simulink model "FOCwithLOAD"  (R2024b)
settings: Solver=FixedStepDiscrete  StartTime=0.0  StopTime=inf  RelTol=1e-3
PreLoadFcn:
  | % 自动加载同目录下的 linear_data.m，确保换机/首次打开可直接更新与编译
  | if ~evalin('base', 'exist(''Ts'',''var'') && exist(''pmsm'',''var'') && exist(''SMRC_I_Vsat_thresh'',''var'')')
  |     mdlDir_ = '';
  |     if bdIsLoaded('FOCwithLOAD'), mdlDir_ = fileparts(get_param('FOCwithLOAD', 'FileName')); end
  |     if isempty(mdlDir_), mdlDir_ = fileparts(which('FOCwithLOAD')); end
  |     if isempty(mdlDir_), mdlDir_ = pwd; end
  |     dataFile_ = fullfile(mdlDir_, 'linear_data.m');
  |     if isfile(dataFile_)
  |         assignin('base', 'linearDataFileTmp_', dataFile_);
  |         evalin('base', 'run(linearDataFileTmp_); clear linearDataFileTmp_');
  |     end
  |     clear mdlDir_ dataFile_
  | end
InitFcn:
  | % 自动加载同目录下的 linear_data.m，确保换机/首次打开可直接更新与编译
  | if ~evalin('base', 'exist(''Ts'',''var'') && exist(''pmsm'',''var'') && exist(''SMRC_I_Vsat_thresh'',''var'')')
  |     mdlDir_ = '';
  |     if bdIsLoaded('FOCwithLOAD'), mdlDir_ = fileparts(get_param('FOCwithLOAD', 'FileName')); end
  |     if isempty(mdlDir_), mdlDir_ = fileparts(which('FOCwithLOAD')); end
  |     if isempty(mdlDir_), mdlDir_ = pwd; end
  |     dataFile_ = fullfile(mdlDir_, 'linear_data.m');
  |     if isfile(dataFile_)
  |         assignin('base', 'linearDataFileTmp_', dataFile_);
  |         evalin('base', 'run(linearDataFileTmp_); clear linearDataFileTmp_');
  |     end
  |     clear mdlDir_ dataFile_
  | end
values from neighbouring files (symbols this model uses):
  a_hat = Kt_eff / (pmsm.J * omega_pu_base)    [linear_data.m]
  ADRC_B0 = 6055    [linear_data.m]
  ADRC_Wc = 3.2e-3    (= 0.0032)    [linear_data.m]
  ADRC_Wo = 30    [linear_data.m]
  alpha_ppc = exp(-lambda_ppc*Ts_speed)    [linear_data.m]
  b_hat = pmsm.B/pmsm.J    [linear_data.m]
  beta1 = single(2.0 * w_o)    [linear_data.m]
  beta2_sat_scale = 0.2    [linear_data.m]
  dataType = 'single'    [linear_data.m]
  gamma_reset = 0.9    [linear_data.m]
  inv_a_hat = 1/double(a_hat)    [linear_data.m]
  k_xi = 55    [linear_data.m]
  Kff = 0.98931745    [linear_data.m]
  lambda_ppc = 45    [linear_data.m]
  P_inf_const = 0.004    [linear_data.m]
  PI_params = mcb_SetControllerParameters(pmsm,inverter,PU_System,T_pwm,Ts,Ts_speed)    [linear_data.m]
  pmsm2 = pmsm    [linear_data.m]
  s_limit_sat = 0.9    [linear_data.m]
  speedRPM2mmps = pmlsm.mmps_per_rpm    [linear_data.m]
  target = mcb_SetProcessorDetails('F28379D',PWM_frequency)    [linear_data.m]
  Ts = T_pwm    (= 5e-05)    [linear_data.m]
  Ts_motor = T_pwm/2    (= 2.5e-05)    [linear_data.m]
  Ts_speed = 1*Ts    (= 5e-05)    [linear_data.m]
  w_o = single(200.0)    [linear_data.m]
  z2_limit = single(100.0)    [linear_data.m]
undefined symbols (not defined in the file or in its folder): DiscIntNeverNeededParam, Down, GPTRIP1SEL, GPTRIP2SEL, innerPI, inverter, inverter2, outerPI, pmlsm, pmsm, Tctr, TZ1, TZ2, Up
libraries: c2802xlib x13, simulink x10, c2837xDlib x6, c280xlib x6, slpidlib x5, svdschedulerlib x4, mcbcontrolslib x4, mcbpositiondecoderlib x2, mcbpmsmnonlinearlib x2, autolibpmsmexterior x2, mcbplantlib x2, svdutilitieslib x1
(part 3 of 5)

== system FOCwithLOAD/Motor1 Speed control/SCI (Code Generation)/Data_Conditioning_Tx ==
  In1 : Inport
  Data_Type_Fixed_Point : Subsystem  VariantControl=~isequal(dataType,'single')
  Data_Type_Float : Subsystem  VariantControl=isequal(dataType, 'single')
  Data_Log : Outport

== system FOCwithLOAD/Motor1 Speed control/SCI (Code Generation)/Data_Logging ==
  note: Fast Serial Data Monitoring (32-bit)
  Data_Log : Inport
  Counter Limited : simulink/Sources/Counter Limited  uplimit=600-1  tsamp=-1
  Data : Subsystem  TreatAsAtomicUnit=on
  End : Subsystem  TreatAsAtomicUnit=on
  If : If  IfExpression=u1 == 0  ElseIfExpressions=u1 == 599
  Merge : Merge  Inputs=3
  Merge1 : Merge  Inputs=3
  Mux : Mux  Inputs=2
  Start : Subsystem  TreatAsAtomicUnit=on
  Width : Width  OutDataTypeMode=All ports same datatype  DataType=uint16
  SCI_Tx : Outport
  wires:
  If/3 -> Data/Action
  Data/1(Data_out) -> Merge/3
  Width/1 -> Data/2(Data_width), Start/2(Data_width), End/2(Data_width)
  Merge/1 -> Mux/1  "SCI_Tx_Data"
  Counter Limited/1 -> If/1
  Start/2(Iteration) -> Merge1/1
  Start/1(Data_out) -> Merge/1
  If/2 -> End/Action
  Merge1/1 -> Mux/2  "SCI_Tx_Iteration"
  If/1 -> Start/Action
  End/1(Data_out) -> Merge/2
  End/2(Iteration) -> Merge1/2
  Data/2(Iteration) -> Merge1/3
  Mux/1 -> SCI_Tx/1
  Data_Log/1 -> Width/1, Start/1(Data), End/1(Data), Data/1(Data)

== system FOCwithLOAD/Motor1 Speed control/SCI (Code Generation)/While Iterator Subsystem ==
  Data : Inport
  Iteration : Inport  Port=2
  Add : Sum  Inputs=+-  OutDataTypeStr=Inherit: Same as first input
  Index Vector : MultiPortSwitch  Inputs=1  SaturateOnIntegerOverflow=off  InputSameDT=off
  SCI Transmit : c280xlib/SCI Transmit  sciModule=A  dataHead=''  dataTail=''  frameSize=1  blockingMode=on  outputStatus=off
  While Iterator : WhileIterator  MaxIters=-1  WhileBlockType=do-while  ShowIterationPort=on  OutputDataType=int16
  wires:
  While Iterator/1 -> Add/2, Index Vector/1
  Data/1 -> Index Vector/2
  Index Vector/1 -> SCI Transmit/1
  Add/1 -> While Iterator/1
  Iteration/1 -> Add/1

== system FOCwithLOAD/Motor1 and Motor2 coupled/Simulation/Load_Friction ==
  spd_rpm : Inport
  Fc_to_Tq : Gain  Gain=pmlsm.F_fric_rated*pmlsm.tau_elec/(2*pi)
  inv_veps : Gain  Gain=1/0.002
  rpm2mps : Gain  Gain=pmlsm.rpm2mps
  tanh_fric : Trigonometry  Operator=tanh
  T_fric : Outport
  wires:
  spd_rpm/1 -> rpm2mps/1
  rpm2mps/1 -> inv_veps/1
  inv_veps/1 -> tanh_fric/1
  tanh_fric/1 -> Fc_to_Tq/1
  Fc_to_Tq/1 -> T_fric/1

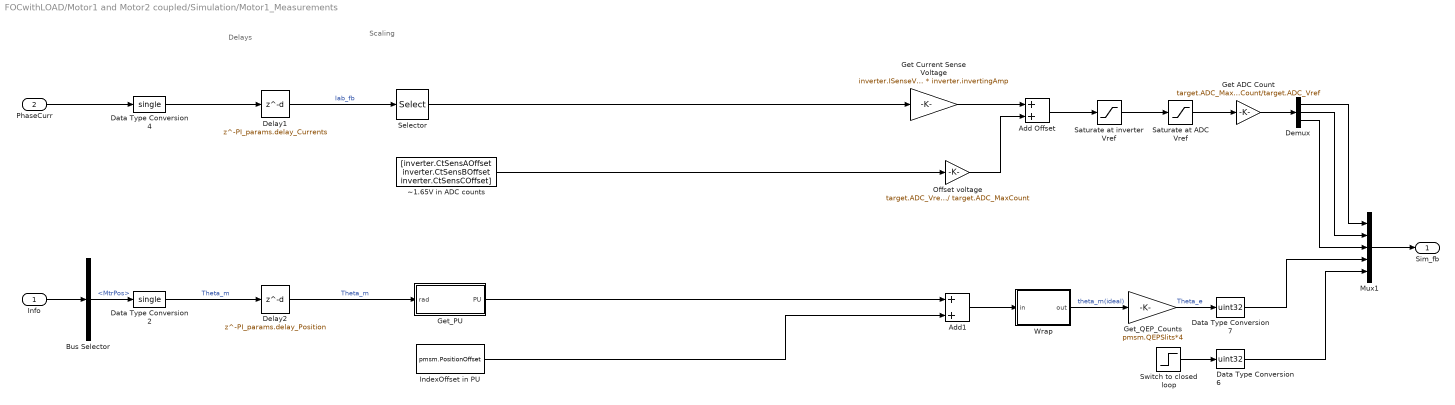
== system FOCwithLOAD/Motor1 and Motor2 coupled/Simulation/Motor1_Measurements ==
  note: Delays
  note: Scaling
  Info : Inport
  PhaseCurr : Inport  Port=2
  Add Offset : Sum  RndMeth=Simplest
  Add1 : Sum  RndMeth=Simplest
  Bus Selector : BusSelector  OutputSignals=MtrPos
  Data Type Conversion2 : DataTypeConversion  OutDataTypeStr=single  RndMeth=Simplest  SaturateOnIntegerOverflow=off
  Data Type Conversion4 : DataTypeConversion  OutDataTypeStr=single  RndMeth=Simplest  SaturateOnIntegerOverflow=off
  Data Type Conversion6 : DataTypeConversion  OutDataTypeStr=uint32  RndMeth=Simplest  SaturateOnIntegerOverflow=off
  Data Type Conversion7 : DataTypeConversion  OutDataTypeStr=uint32  RndMeth=Simplest  SaturateOnIntegerOverflow=off
  Delay1 : Delay  DelayLength=PI_params.delay_Currents
  Delay2 : Delay  DelayLength=PI_params.delay_Position
  Demux : Demux  Outputs=3
  Get ADC Count : Gain  Gain=target.ADC_MaxCount/target.ADC_Vref  OutMin=0  OutMax=target.ADC_MaxCount  OutDataTypeStr=uint32  RndMeth=Simplest
  Get Current Sense Voltage : Gain  Gain=inverter.ISenseVoltPerAmp * inverter.invertingAmp  RndMeth=Simplest  OutDataTypeStr=Inherit: Same as input
  "Get_PU " : Subsystem
  Get_QEP_Counts : Gain  Gain=pmsm.QEPSlits*4  OutDataTypeStr=uint32  RndMeth=Simplest
  IndexOffset in PU : Constant  Value=pmsm.PositionOffset  OutDataTypeStr=single  SampleTime=-1
  Mux1 : Mux  Inputs=5
  Offset voltage : Gain  Gain=target.ADC_Vref / target.ADC_MaxCount  RndMeth=Simplest
  Saturate at ADC Vref : Saturate  UpperLimit=target.ADC_Vref  LowerLimit=0
  Saturate at inverter Vref : Saturate  UpperLimit=inverter.ISenseVref  LowerLimit=0
  Selector : Selector  InputPortWidth=3  IndexOptions=Index vector (dialog)  Indices=[1 2 3]  OutputSizes=1
  "Switch to closed loop " : Step  Time=0.1  SampleTime=Ts_motor
  Wrap : Subsystem
  ~1.65V in ADC counts : Constant  Value="[inverter.CtSensAOffset inverter.CtSensBOffset  inverter.CtSensCOffset]"  OutDataTypeStr=uint16  SampleTime=-1
  Sim_fb : Outport  VectorParamsAs1DForOutWhenUnconnected=off
  wires:
  "Switch to closed loop "/1 -> Data Type Conversion6/1
  Data Type Conversion6/1 -> Mux1/5
  Data Type Conversion7/1 -> Mux1/4
  IndexOffset in PU/1 -> Add1/2
  Get_QEP_Counts/1 -> Data Type Conversion7/1  "Theta_e"
  "Get_PU "/1(PU) -> Add1/1
  Wrap/1(out) -> Get_QEP_Counts/1  "theta_m(ideal)"
  Delay2/1 -> "Get_PU "/1(rad)  "Theta_m"
  Add1/1 -> Wrap/1(in)
  Data Type Conversion2/1 -> Delay2/1  "Theta_m"
  Demux/2 -> Mux1/2
  Mux1/1 -> Sim_fb/1
  Demux/1 -> Mux1/1
  Bus Selector/1 -> Data Type Conversion2/1  "<MtrPos>"
  Info/1 -> Bus Selector/1
  PhaseCurr/1 -> Data Type Conversion4/1
  Data Type Conversion4/1 -> Delay1/1
  Delay1/1 -> Selector/1  "Iab_fb"
  Saturate at ADC Vref/1 -> Get ADC Count/1
  Offset voltage/1 -> Add Offset/2
  Get ADC Count/1 -> Demux/1
  Saturate at inverter Vref/1 -> Saturate at ADC Vref/1
  Add Offset/1 -> Saturate at inverter Vref/1
  Get Current Sense Voltage/1 -> Add Offset/1
  ~1.65V in ADC counts/1 -> Offset voltage/1
  Demux/3 -> Mux1/3
  Selector/1 -> Get Current Sense Voltage/1

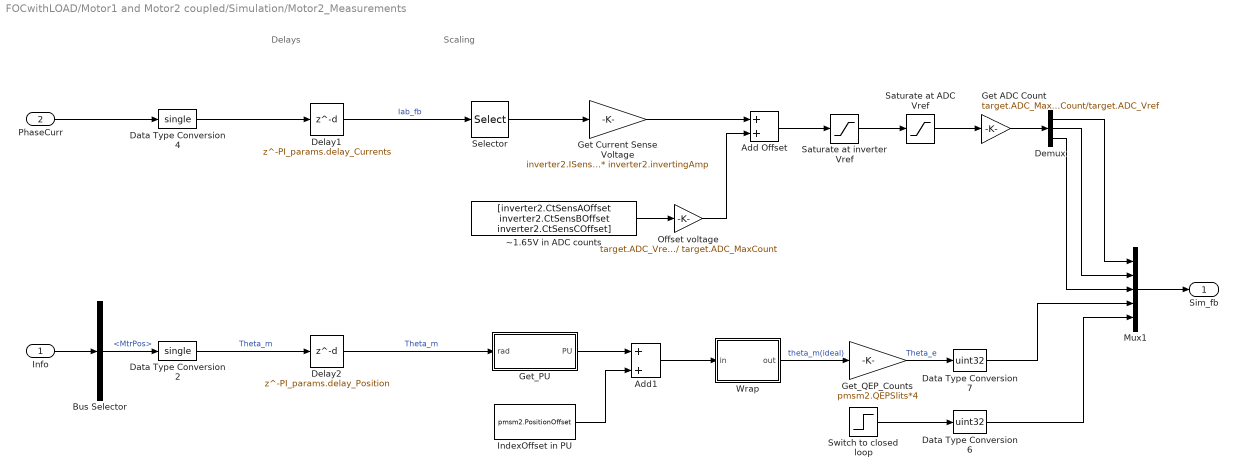
== system FOCwithLOAD/Motor1 and Motor2 coupled/Simulation/Motor2_Measurements ==
  note: Scaling
  note: Delays
  Info : Inport
  PhaseCurr : Inport  Port=2
  Add Offset : Sum  RndMeth=Simplest
  Add1 : Sum  RndMeth=Simplest
  Bus Selector : BusSelector  OutputSignals=MtrPos
  Data Type Conversion2 : DataTypeConversion  OutDataTypeStr=single  RndMeth=Simplest  SaturateOnIntegerOverflow=off
  Data Type Conversion4 : DataTypeConversion  OutDataTypeStr=single  RndMeth=Simplest  SaturateOnIntegerOverflow=off
  Data Type Conversion6 : DataTypeConversion  OutDataTypeStr=uint32  RndMeth=Simplest  SaturateOnIntegerOverflow=off
  Data Type Conversion7 : DataTypeConversion  OutDataTypeStr=uint32  RndMeth=Simplest  SaturateOnIntegerOverflow=off
  Delay1 : Delay  DelayLength=PI_params.delay_Currents
  Delay2 : Delay  DelayLength=PI_params.delay_Position
  Demux : Demux  Outputs=3
  Get ADC Count : Gain  Gain=target.ADC_MaxCount/target.ADC_Vref  OutMin=0  OutMax=target.ADC_MaxCount  OutDataTypeStr=uint32  RndMeth=Simplest
  Get Current Sense Voltage : Gain  Gain=inverter2.ISenseVoltPerAmp * inverter2.invertingAmp  RndMeth=Simplest  OutDataTypeStr=Inherit: Same as input
  "Get_PU " : Subsystem
  Get_QEP_Counts : Gain  Gain=pmsm2.QEPSlits*4  OutDataTypeStr=uint32  RndMeth=Simplest
  IndexOffset in PU : Constant  Value=pmsm2.PositionOffset  OutDataTypeStr=single  SampleTime=-1
  Mux1 : Mux  Inputs=5
  Offset voltage : Gain  Gain=target.ADC_Vref / target.ADC_MaxCount  RndMeth=Simplest
  Saturate at ADC Vref : Saturate  UpperLimit=target.ADC_Vref  LowerLimit=0
  Saturate at inverter Vref : Saturate  UpperLimit=inverter2.ISenseVref  LowerLimit=0
  Selector : Selector  InputPortWidth=3  IndexOptions=Index vector (dialog)  Indices=[1 2 3]  OutputSizes=1
  "Switch to closed loop " : Step  Time=0.1  SampleTime=Ts_motor
  Wrap : Subsystem
  ~1.65V in ADC counts : Constant  Value=[inverter2.CtSensAOffset inverter2.CtSensBOffset inverter2.CtSensCOffset]  OutDataTypeStr=uint16  SampleTime=-1
  Sim_fb : Outport  VectorParamsAs1DForOutWhenUnconnected=off
  wires:
  Delay1/1 -> Selector/1  "Iab_fb"
  Data Type Conversion4/1 -> Delay1/1
  PhaseCurr/1 -> Data Type Conversion4/1
  Info/1 -> Bus Selector/1
  Bus Selector/1 -> Data Type Conversion2/1  "<MtrPos>"
  Demux/1 -> Mux1/1
  Mux1/1 -> Sim_fb/1
  Demux/2 -> Mux1/2
  Data Type Conversion2/1 -> Delay2/1  "Theta_m"
  Add1/1 -> Wrap/1(in)
  Delay2/1 -> "Get_PU "/1(rad)  "Theta_m"
  Wrap/1(out) -> Get_QEP_Counts/1  "theta_m(ideal)"
  "Get_PU "/1(PU) -> Add1/1
  Get_QEP_Counts/1 -> Data Type Conversion7/1  "Theta_e"
  IndexOffset in PU/1 -> Add1/2
  Data Type Conversion7/1 -> Mux1/4
  Data Type Conversion6/1 -> Mux1/5
  "Switch to closed loop "/1 -> Data Type Conversion6/1
  Saturate at ADC Vref/1 -> Get ADC Count/1
  Offset voltage/1 -> Add Offset/2
  Selector/1 -> Get Current Sense Voltage/1
  Get ADC Count/1 -> Demux/1
  Saturate at inverter Vref/1 -> Saturate at ADC Vref/1
  Add Offset/1 -> Saturate at inverter Vref/1
  Get Current Sense Voltage/1 -> Add Offset/1
  ~1.65V in ADC counts/1 -> Offset voltage/1
  Demux/3 -> Mux1/3

== system FOCwithLOAD/Motor1 and Motor2 coupled/Simulation/Mtr1 Inverter ==
  Duty_abc : Inport
  Average-Value Inverter : mcbplantlib/Average-Value Inverter
  Constant2 : Constant  Value=inverter.V_dc  OutDataTypeStr=single
  Data Type Conversion1 : DataTypeConversion  OutDataTypeStr=single  RndMeth=Simplest  SaturateOnIntegerOverflow=off
  Rate Transition3 : RateTransition  Integrity=off  OutPortSampleTime=Ts_inverter
  Vabc : Outport  VectorParamsAs1DForOutWhenUnconnected=off
  wires:
  Constant2/1 -> Average-Value Inverter/2
  Data Type Conversion1/1 -> Rate Transition3/1
  Average-Value Inverter/1 -> Vabc/1
  Duty_abc/1 -> Data Type Conversion1/1
  Rate Transition3/1 -> Average-Value Inverter/1

== system FOCwithLOAD/Motor1 and Motor2 coupled/Simulation/Mtr2 Inverter ==
  Duty_abc : Inport
  Average-Value Inverter : mcbplantlib/Average-Value Inverter
  Constant2 : Constant  Value=inverter2.V_dc  OutDataTypeStr=single
  Data Type Conversion1 : DataTypeConversion  OutDataTypeStr=single  RndMeth=Simplest  SaturateOnIntegerOverflow=off
  Rate Transition3 : RateTransition  Integrity=off  OutPortSampleTime=Ts_inverter
  Vabc : Outport  VectorParamsAs1DForOutWhenUnconnected=off
  wires:
  Data Type Conversion1/1 -> Rate Transition3/1
  Average-Value Inverter/1 -> Vabc/1
  Duty_abc/1 -> Data Type Conversion1/1
  Rate Transition3/1 -> Average-Value Inverter/1
  Constant2/1 -> Average-Value Inverter/2

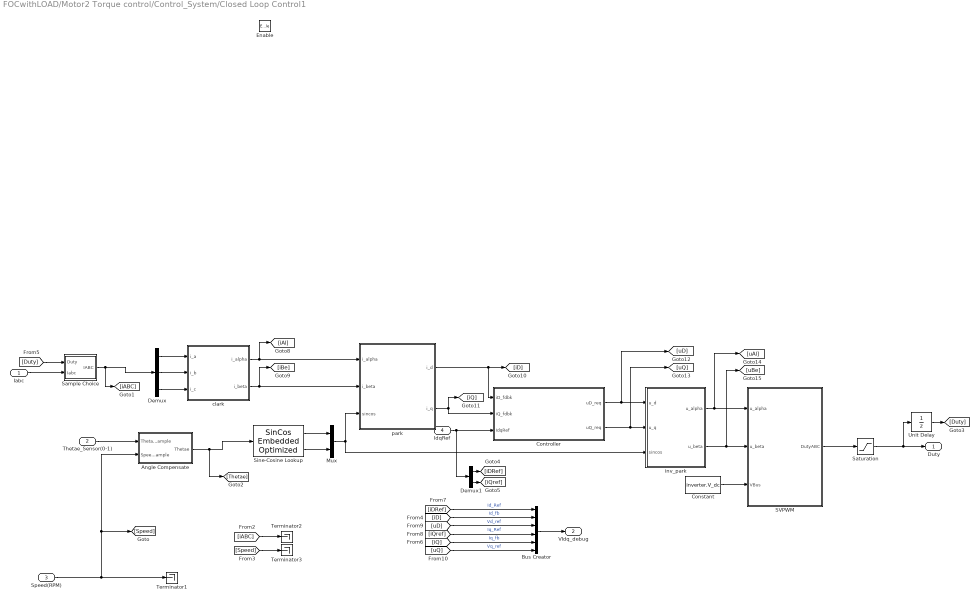
== system FOCwithLOAD/Motor2 Torque control/Control_System/Closed Loop Control1 ==
  Iabc : Inport
  Thetae_Sensor(0-1) : Inport  Port=2
  Speed(RPM) : Inport  Port=3
  IdqRef : Inport  Port=4
  Enable : EnablePort
  Angle Compensate : Subsystem
  Bus Creator : BusCreator  Inputs=6
  Constant : Constant  Value=inverter.V_dc  OutDataTypeStr=single
  Controller : Subsystem
  Demux : Demux  Outputs=3
  Demux1 : Demux  Outputs=2
  Mux : Mux  Inputs=2
  SVPWM : Subsystem
      mask Display:
      | port_label('input',1,'u_{\alpha}','texmode','on');
      | port_label('input',2,'u_{\beta}','texmode','on');
      | port_label('input',3,'V_{Bus}','texmode','on');
      | 
      | port_label('output',1,'Duty_{ABC}','texmode','on');
      | 
      | fprintf('SVPWM');
  Sample Choice : Subsystem
  Saturation : Saturate  UpperLimit=1  LowerLimit=0
  Sine-Cosine Lookup : mcbcontrolslib/SinCos Embedded Optimized  LabelModeActiveChoice=MCB_Sin  OptforProc=off  ApproximationMethod=None  UserApproxMethod=Lookup  ApproxStatus=None  InterpMethod=Linear point-slope  NumberOfDataPoints=16  NumberOfIterations=11  RemoveProtectionAgainstOutOfRangeInput=off  TableDataTypeStr=Inherit: Inherit via input  AngleInput=Per-unit  ThetaDataType=single  N_points=1024  DatatypeInput=Inherit from input  Datatype=Inherit: Same as input
  Terminator1 : Terminator
  Terminator2 : Terminator
  Terminator3 : Terminator
  Unit Delay : UnitDelay  SampleTime=-1  HasFrameUpgradeWarning=on
  clark : Subsystem  TreatAsAtomicUnit=on
      mask Display:
      | port_label('input',1,'a','texmode','on');
      | port_label('input',2,'b','texmode','on');
      | port_label('input',3,'c','texmode','on');
      | 
      | port_label('output',1,'\alpha','texmode','on');
      | port_label('output',2,'\beta','texmode','on');
      | 
      | fprintf('Clark');
  inv_park : Subsystem
      mask Display:
      | port_label('input', 1, 'd', 'texmode', 'on');
      | port_label('input', 2, 'q', 'texmode', 'on');
      | port_label('input', 3, 'sin\theta_e cos\theta_e', 'texmode', 'on');
      | port_label('output', 1, '\alpha', 'texmode', 'on');
      | port_label('output', 2, '\beta', 'texmode', 'on');
      | fprintf('Inverse Park')
  park : Subsystem  TreatAsAtomicUnit=on
      mask Display:
      | port_label('input',1,'\alpha','texmode','on');
      | port_label('input',2,'\beta','texmode','on');
      | port_label('input',3,'sin\theta_e cos\theta_e','texmode','on');
      | 
      | port_label('output',1,'d','texmode','on');
      | port_label('output',2,'q','texmode','on');
      | 
      | fprintf('Park');
  Duty : Outport
  VIdq_debug : Outport  Port=2  VectorParamsAs1DForOutWhenUnconnected=off
  wires:
  inv_park/2(u_beta) -> [uBe], SVPWM/2(u_beta)
  Saturation/1 -> Unit Delay/1, Duty/1
  Demux/2 -> clark/2(i_b)
  Demux/3 -> clark/3(i_c)
  Mux/1 -> inv_park/3(sincos), park/3(sincos)
  Controller/2(uQ_req) -> inv_park/2(u_q), [uQ]
  SVPWM/1(DutyABC) -> Saturation/1
  park/1(i_d) -> [iD], Controller/1(iD_fdbk)
  Controller/1(uD_req) -> inv_park/1(u_d), [uD]
  clark/1(i_alpha) -> [iAl], park/1(i_alpha)
  clark/2(i_beta) -> [iBe], park/2(i_beta)
  inv_park/1(u_alpha) -> [uAl], SVPWM/1(u_alpha)
  park/2(i_q) -> Controller/2(iQ_fdbk), [iQ]
  Demux/1 -> clark/1(i_a)
  Sine-Cosine Lookup/1 -> Mux/1
  Sine-Cosine Lookup/2 -> Mux/2
  [Duty] -> Sample Choice/1(Duty)
  Unit Delay/1 -> [Duty]
  Constant/1 -> SVPWM/3(VBus)
  Speed(RPM)/1 -> Terminator1/1, Angle Compensate/2(SpeedSample), [Speed]
  Thetae_Sensor(0-1)/1 -> Angle Compensate/1(ThetaeSample)
  Angle Compensate/1(Thetae) -> [Thetae], Sine-Cosine Lookup/1
  Iabc/1 -> Sample Choice/2(Iabc)
  Sample Choice/1(IABC) -> Demux/1, [iABC]
  [iABC] -> Terminator2/1
  [Speed] -> Terminator3/1
  IdqRef/1 -> Demux1/1, Controller/3(IdqRef)
  [iDRef] -> Bus Creator/1  "Id_Ref"
  [iD] -> Bus Creator/2  "Id_fb"
  Bus Creator/1 -> VIdq_debug/1
  [uQ] -> Bus Creator/6  "Vq_ref"
  [uD] -> Bus Creator/3  "Vd_ref"
  [iQ] -> Bus Creator/5  "Iq_fb"
  [iQref] -> Bus Creator/4  "Iq_Ref"
  Demux1/1 -> [iDRef]
  Demux1/2 -> [iQref]

== system FOCwithLOAD/Motor2 Torque control/HW_Inputs/Sensor Driver Blocks (codegen) ==
  Sim : Inport
  ADC_A_IN4 : c2802xlib/ADC  Priority=1  blkParamProc=C2000_Type4  ADCModule=A  samplingMode=Single sample mode  ADCResolution=12-bit (Single-ended input)  useSOC1=SOC1  useSOC2=SOC0_SOC1  SOCAcquisitionWindow=30  SOCTriggerSource=ePWM4_ADCSOCA  SOCInterruptTrigger=No ADCINT  Ts=-1  dType=uint16  postInterrupt=off  interruptSel=ADCINT1  ADCINTContinuous=on  endma=off  chdma=1  conv1=ADCINA0  conv2=ADCINA0 and ADCINB0  conv1_Type4=ADCIN4  conv2_Type4=ADCIN0 and ADCIN1
  ADC_A_IN4_u32 : DataTypeConversion  OutDataTypeStr=uint32  SaturateOnIntegerOverflow=off  RndMeth=Floor
  ADC_B_IN4 : c2802xlib/ADC  Priority=2  blkParamProc=C2000_Type4  ADCModule=B  samplingMode=Single sample mode  ADCResolution=12-bit (Single-ended input)  useSOC1=SOC1  useSOC2=SOC0_SOC1  SOCAcquisitionWindow=30  SOCTriggerSource=ePWM4_ADCSOCA  SOCInterruptTrigger=No ADCINT  Ts=-1  dType=uint16  postInterrupt=off  interruptSel=ADCINT1  ADCINTContinuous=on  endma=off  chdma=1  conv1=ADCINA0  conv2=ADCINA0 and ADCINB0  conv1_Type4=ADCIN4  conv2_Type4=ADCIN0 and ADCIN1
  ADC_B_IN4_u32 : DataTypeConversion  OutDataTypeStr=uint32  SaturateOnIntegerOverflow=off  RndMeth=Floor
  ADC_C_IN4 : c2802xlib/ADC  Priority=3  blkParamProc=C2000_Type4  ADCModule=C  samplingMode=Single sample mode  ADCResolution=12-bit (Single-ended input)  useSOC1=SOC1  useSOC2=SOC0_SOC1  SOCAcquisitionWindow=30  SOCTriggerSource=ePWM4_ADCSOCA  SOCInterruptTrigger=No ADCINT  Ts=-1  dType=uint16  postInterrupt=on  interruptSel=ADCINT1  ADCINTContinuous=on  endma=off  chdma=1  conv1=ADCINA0  conv2=ADCINA0 and ADCINB0  conv1_Type4=ADCIN4  conv2_Type4=ADCIN0 and ADCIN1
  ADC_C_IN4_u32 : DataTypeConversion  OutDataTypeStr=uint32  SaturateOnIntegerOverflow=off  RndMeth=Floor
  Mux1 : Mux  Inputs=5
  Terminator : Terminator
  eQEP2 for PMSM2 : c280xlib/eQEP  Priority=0  useModule=eQEP2  pcInputmode=Quadrature-count  externalClockrate=2x resolution: Count the rising/falling edge  swapPolarityselection=Counterclockwise  qdfOutputport=off  qapPolarityselection=off  qbpPolarityselection=off  qipPolarityselection=off  qspPolarityselection=off  igatePolarityselection=off  sampleTime=-1  pcOutputport=on  pcMaximumvalue=2^32-1  indexInitializationcheck=off  indexInitializationevent=Rising edge  strobeInitializationcheck=off  strobeInitializationevent=Rising edge  softwareInitializationcheck=off  softwareInitializationsource=Set to init value at start up  softwareInitializationmode=on  pcInitialvalue=0  pcResetmode=Reset on the maximum position  ieloutputport=on  indexEventlatch=Rising edge  seloutputport=off  strobeEventlatch=Rising edge  pcefOutputport=off  enableEqepcapture=off  qctmrOutputport=off  qcprdOutputport=off  captureTimerprescaler=128  upEventprescaler=128  overflowErrorflag=off  directionErrorflag=off  captureTimerposition=On position counter read  unitTimerperiod=100000000  captureTimerlatch=off  capturePeriodlatch=off  positionCounterlatch=off  soenPolarityselection=off  spselPolarityselection=Index pin is used for sync output  compareValuesource=Specify via dialog  shadowMode=Load on QPOSCNT=0  compareValue=4294967295  syncOutputwidth=1  polaritySyncoutput=Active high  watchdogEnable=off  watchdogTimer=65535  outport1Datatype=uint32  outport2Datatype=auto  outport3Datatype=auto  outport4Datatype=auto  outport5Datatype=auto  outport6Datatype=auto  outport7Datatype=auto  outport8Datatype=auto  outport9Datatype=auto  outport10Datatype=auto  outport11Datatype=auto  outport12Datatype=auto  eqepinterrupt_pce=off  eqepinterrupt_qpe=off  eqepinterrupt_qdc=off  eqepinterrupt_wto=off  eqepinterrupt_pcu=off  eqepinterrupt_pco=off  eqepinterrupt_pcr=off  eqepinterrupt_pcm=off  eqepinterrupt_sel=off  eqepinterrupt_iel=off  eqepinterrupt_uto=off  pheOutputport=off  watchdogOutputport=off  outport13Datatype=auto  outport14Datatype=auto
      settings: LibrarySourceBlock=c28002xlib/eQEP
  read_qep32 : CFunction  OutputCode=|  CodegenOutputCode=|
      OutputCode=|
      | /* 32-bit read: legacy c280xqep truncates QPOSCNT to uint16 */
      | y1 = (uint32_T)EQep2Regs.QPOSCNT;
      | y2 = (uint32_T)EQep2Regs.QPOSILAT;
      CodegenOutputCode=|
      | /* 32-bit read: legacy c280xqep truncates QPOSCNT to uint16 */
      | y1 = (uint32_T)EQep2Regs.QPOSCNT;
      | y2 = (uint32_T)EQep2Regs.QPOSILAT;
  term_qep2_1 : Terminator
  term_qep2_2 : Terminator
  Out : Outport
  wires:
  Mux1/1 -> Out/1
  Sim/1 -> Terminator/1
  ADC_A_IN4/1 -> ADC_A_IN4_u32/1
  ADC_A_IN4_u32/1 -> Mux1/1
  ADC_B_IN4/1 -> ADC_B_IN4_u32/1
  ADC_B_IN4_u32/1 -> Mux1/2
  ADC_C_IN4/1 -> ADC_C_IN4_u32/1
  ADC_C_IN4_u32/1 -> Mux1/3
  eQEP2 for PMSM2/1 -> term_qep2_1/1
  eQEP2 for PMSM2/2 -> term_qep2_2/1
  read_qep32/1 -> Mux1/4
  read_qep32/2 -> Mux1/5

== system FOCwithLOAD/Motor2 Torque control/HW_Inputs/Sensor Driver Blocks (sim) ==
  Sim : Inport
  Out : Outport
  wires:
  Sim/1 -> Out/1

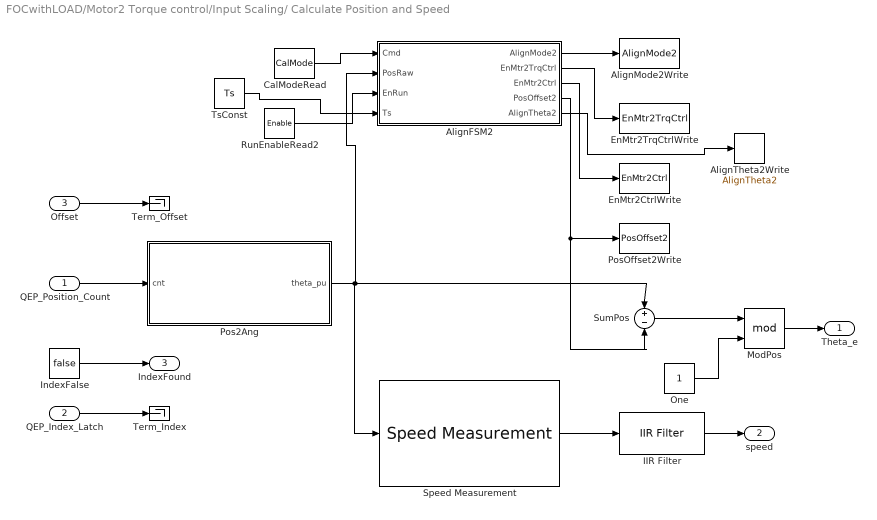
== system FOCwithLOAD/Motor2 Torque control/Input Scaling/ Calculate Position and Speed ==
  QEP_Position_Count : Inport
  QEP_Index_Latch : Inport  Port=2
  Offset : Inport  Port=3
  AlignFSM2 : MATLAB Function  TreatAsAtomicUnit=on
  AlignMode2Write : DataStoreWrite  DataStoreName=AlignMode2  IndexOptions=Index vector (dialog)  Indices=1  OutputSizes=1
  AlignTheta2Write : DataStoreWrite  DataStoreName=AlignTheta2  IndexOptions=Index vector (dialog)  Indices=1  OutputSizes=1
  CalModeRead : DataStoreRead  DataStoreName=CalMode  IndexOptions=Index vector (dialog)  Indices=1  OutputSizes=1
  EnMtr2CtrlWrite : DataStoreWrite  DataStoreName=EnMtr2Ctrl  IndexOptions=Index vector (dialog)  Indices=1  OutputSizes=1
  EnMtr2TrqCtrlWrite : DataStoreWrite  DataStoreName=EnMtr2TrqCtrl  IndexOptions=Index vector (dialog)  Indices=1  OutputSizes=1
  IIR Filter : mcbcontrolslib/IIR Filter  VariantControl=Low Pass Filter  VariantSelect=Low-pass  FilterConstantInputType=Specify via dialog  Filter_constant=0.1  advancedSettings=on  Ts=50e-6  cutOff_freq=353.6777
  IndexFalse : Constant  Value=false  OutDataTypeStr=boolean
  ModPos : Math  Operator=mod
  One : Constant  OutDataTypeStr=single
  Pos2Ang : MATLAB Function  TreatAsAtomicUnit=on
  PosOffset2Write : DataStoreWrite  DataStoreName=PosOffset2  IndexOptions=Index vector (dialog)  Indices=1  OutputSizes=1
  RunEnableRead2 : DataStoreRead  DataStoreName=Enable  IndexOptions=Index vector (dialog)  Indices=1  OutputSizes=1
  Speed Measurement : mcbpositiondecoderlib/Speed Measurement  PositionUnit=Per unit  PositionScalingDatatype=uint32  SpeedCalculationMode=Time interval for speed calculation  SampleTimeAsync=Ts  MaximumApplicationSpeed=6000  SpeedResolution=5e-6  DelayLength=200  MaximumMeasurableSpeed=2999  MeasurableSpeedResolution=1.397e-06  SpeedUnit=RPM  PerUnitSpeed=3000  SpeedDataType=dataType
  SumPos : Sum  Inputs=+-
  Term_Index : Terminator
  Term_Offset : Terminator
  TsConst : Constant  Value=Ts  OutDataTypeStr=single
  Theta_e : Outport  VectorParamsAs1DForOutWhenUnconnected=off
  speed : Outport  Port=2  VectorParamsAs1DForOutWhenUnconnected=off
  IndexFound : Outport  Port=3
  wires:
  CalModeRead/1 -> AlignFSM2/1(Cmd)
  ModPos/1 -> Theta_e/1
  Offset/1 -> Term_Offset/1
  QEP_Position_Count/1 -> Pos2Ang/1(cnt)
  QEP_Index_Latch/1 -> Term_Index/1
  IndexFalse/1 -> IndexFound/1
  AlignFSM2/1(AlignMode2) -> AlignMode2Write/1
  Pos2Ang/1(theta_pu) -> SumPos/1, AlignFSM2/2(PosRaw), Speed Measurement/1
  AlignFSM2/2(EnMtr2TrqCtrl) -> EnMtr2TrqCtrlWrite/1
  AlignFSM2/3(EnMtr2Ctrl) -> EnMtr2CtrlWrite/1
  AlignFSM2/4(PosOffset2) -> SumPos/2, PosOffset2Write/1
  Speed Measurement/1 -> IIR Filter/1
  SumPos/1 -> ModPos/1
  One/1 -> ModPos/2
  IIR Filter/1 -> speed/1
  RunEnableRead2/1 -> AlignFSM2/3(EnRun)
  AlignFSM2/5(AlignTheta2) -> AlignTheta2Write/1
  TsConst/1 -> AlignFSM2/4(Ts)

== system FOCwithLOAD/Motor2 Torque control/Input Scaling/Calculate Phase Currents ==
  Ia_ADC : Inport
  Ib_ADC : Inport  Port=2
  Ic_ADC : Inport  Port=3
  Add : Sum  Inputs=-+
  Data Store Read1 : DataStoreRead  DataStoreName=IaOffset_motor2  IndexOptions=Index vector (dialog)  Indices=1  OutputSizes=1
  Data Store Read2 : DataStoreRead  DataStoreName=IbOffset_motor2  IndexOptions=Index vector (dialog)  Indices=1  OutputSizes=1
  Data Store Read4 : DataStoreRead  DataStoreName=IcOffset_motor2  IndexOptions=Index vector (dialog)  Indices=1  OutputSizes=1
  Data Type Conversion : DataTypeConversion  OutDataTypeStr=int32  ConvertRealWorld=Stored Integer (SI)  RndMeth=Simplest  SaturateOnIntegerOverflow=off
  Data_Type : Subsystem  Variant=on
  Inverting / Non-inverting Current measurement amplifieer : Gain  Gain=inverter2.invertingAmp  RndMeth=Simplest  OutDataTypeStr=Inherit: Same as input
  Mux : Mux  Inputs=3
  Mux1 : Mux  Inputs=3
  Iabc_meas_Real : Outport  VectorParamsAs1DForOutWhenUnconnected=off
  wires:
  Data Type Conversion/1 -> Add/2
  Data_Type/1(Iabc_meas_Real) -> Inverting / Non-inverting Current measurement amplifieer/1
  Ia_ADC/1 -> Mux/1
  Ib_ADC/1 -> Mux/2
  Mux/1 -> Data Type Conversion/1
  Data Store Read1/1 -> Mux1/1
  Data Store Read2/1 -> Mux1/2
  Mux1/1 -> Add/1
  Add/1 -> Data_Type/1(In1)
  Ic_ADC/1 -> Mux/3
  Data Store Read4/1 -> Mux1/3
  Inverting / Non-inverting Current measurement amplifieer/1 -> Iabc_meas_Real/1

== system FOCwithLOAD/Motor2 Torque control/Inverter/Code Generation ==
  note: for inverter connected with LaunchXL-28379D
  note: System Outputs
  Inverter Signals : Inport
  Constant : Constant  Value=inverter2.EnableLogic
  Demux : Demux
  Demux1 : Demux  Outputs=3
  Ground : Ground
  Ground1 : Ground
  Ground2 : Ground
  Inverter2 Enable : c2837xDlib/Digital Output  GPIO_Number=GPIO8~GPIO15  GPIO_Bit0=off  GPIO_BIT0_Toggle=off  GPIO_Bit1=off  GPIO_BIT1_Toggle=off  GPIO_Bit2=off  GPIO_BIT2_Toggle=off  GPIO_Bit3=off  GPIO_BIT3_Toggle=off  GPIO_Bit4=off  GPIO_BIT4_Toggle=off  GPIO_Bit5=off  GPIO_BIT5_Toggle=off  GPIO_Bit6=on  GPIO_BIT6_Toggle=off  GPIO_Bit7=off  GPIO_BIT7_Toggle=off
  Mux : Mux  Inputs=3
  Mux1 : Mux  Inputs=3
  Mux2 : Mux  Inputs=3
  NOT : Logic  Operator=NOT  IconShape=distinctive  AllPortsSameDT=off  OutDataTypeStr=boolean
  Scale_to_PWM_Counter_PRD : Gain  Gain=target.PWM_Counter_Period  OutDataTypeStr=uint16  RndMeth=Simplest
  Switch : Switch  Criteria=u2 > Threshold  SaturateOnIntegerOverflow=off  InputSameDT=off
  Switch1 : Switch  Threshold=0.5  SaturateOnIntegerOverflow=off  InputSameDT=off
  ePWM4 : c2802xlib/ePWM  PwmType=C2000_Type4  useModule=ePWM4  ePWMxLINKTBPRD=Not Linked  periodUnits=Clock cycles  timerSource=Specify via dialog  timerPeriod_clk=target.PWM_Counter_Period  timerPeriod_sec=0.0001  tbshadow=Counter equals to zero  countingMode=Up-Down  phaseActiveEnable=Set counter to phase value specified via dialog  phaseDirection=Count down after sync  phaseActive=target.PWM_Counter_Period  synchronizationEnable=off  dcaevt1Sync=off  dcbevt1Sync=off  synchronizationOption=Pass through (EPWMxSYNCI or SWFSYNC)  dcbevt1SyncOut=off  dcaevt1SyncOut=off  cmpdSyncOut=off  cmpcSyncOut=off  cmpbSyncOut=off  zeroSyncOut=off  swfSyncOut=on  perSynchronizationOption=Counter equals to period (CTR=PRD)  clockPrescale=1  HSclockPrescale=1  enswap=off  ePWMxAStatus=on  ePWMxAactionLogic1=Do nothing  ePWMxAactionLogic2=Do nothing  ePWMxAactionLogic3=Clear  ePWMxAactionLogic4=Set  ePWMxAactionLogic5=Do nothing  ePWMxAactionLogic6=Do nothing  ePWMxACSFenable=off  ePWMxACSFvalue=Forcing disable  ePWMxASFreload=Zero  ePWMxBStatus=off  ePWMxBactionLogic1=Set  ePWMxBactionLogic2=Clear  ePWMxBactionLogic3=Do nothing  ePWMxBactionLogic4=Do nothing  ePWMxBactionLogic5=Clear  ePWMxBactionLogic6=Set  ePWMxBCSFenable=off  ePWMxBCSFvalue=Forcing disable  ePWMxBSFreload=Zero  ePWNxBOutWay=off  ePWMxLINKCMPA=Not Linked  CMPAUnits=Clock cycles  CMPASource=Input port  CMPAValue_per=50  CMPAValue_clk=floor(target.PWM_Counter_Period/2)  enCMPAshadow=Counter equals to zero (CTR=Zero)  ePWMxLINKCMPB=Not Linked  CMPBUnits=Clock cycles  CMPBSource=Specify via dialog  CMPBValue_per=50  CMPBValue_clk=floor(target.PWM_Counter_Period/2)  enCMPBshadow=Counter equals to zero (CTR=Zero)  ePWMxLINKCMPC=Not Linked  CMPCUnits=Clock cycles  CMPCSource=Specify via dialog  CMPCValue_per=50  CMPCValue_clk=32000  enCMPCshadow=Counter equals to zero (CTR=Zero)  ePWMxLINKCMPD=Not Linked  CMPDUnits=Clock cycles  CMPDSource=Specify via dialog  CMPDValue_per=50  CMPDValue_clk=32000  enCMPDshadow=Counter equals to zero (CTR=Zero)  enableDBePWMxA=on  enableDBePWMxB=on  enhalfcycle=off  DBpolarity=Active high complementary (AHC)  DBedgeDelay=Positive  DBSource_ePWMxA=ePWMxA  DBSource_ePWMxB=ePWMxA  DBPeriodUnits=Clock cycles  DBperiodSource=Specify via dialog  REDperiod=10  FEDperiod=10  REDperiod_sec=0  FEDperiod_sec=0  LoadModeDBRED=Immediate without using shadow  LoadModeDBFED=Immediate without using shadow  adcstartModuleA=on  adcrequestEventA=First event  adcstartEventA=Digital Compare Module A Event 1 start of conversion (DCAEVT1.soc)  adcstartEventA_type2=Counter equals to period (CTR=PRD)  adcstartModuleB=off  adcrequestEventB=First event  adcstartEventB=Counter equals to zero (CTR=Zero)  adcstartEventB_type2=Counter equals to zero (CTR=Zero)  intEn=off  intPrd=First event  intSel=Counter equals to zero (CTR=Zero)  intSel_type2=Counter equals to zero (CTR=Zero)  hrpe=off  enHRPWM=off  HRPWM_LoadMode=Counter equals to period (CTR=PRD)  HRPWM_CTLMode=Duty or Period control mode  HRPWM_EDGMode=Both edge  hrpeb=off  enHRPWMB=off  HRPWM_LoadModeB=Counter equals to zero (CTR=ZERO)  HRPWM_CTLModeB=Duty or Period control mode  HRPWM_EDGModeB=Both edge  enHRDBRED=off  enHRDBFED=off  enSFO=on  enautoconv=on  chopperEnable=off  chopperFrequency=1  chopperFirstwidth=1  chopperDuty=12.5%  tripZonesource=Specify via dialog  tzselOSHT1=off  tzselOSHT2=off  tzselOSHT3=off  tzselOSHT4=off  tzselOSHT5=off  tzselOSHT6=off  tzselOSHDCAEV1=off  tzselOSHDCBEV1=off  tzselCBC1=off  tzselCBC2=off  tzselCBC3=off  tzselCBC4=off  tzselCBC5=off  tzselCBC6=off  tzselCBCDCAEV2=off  tzselCBCDCBEV2=off  enTzOstIntr=off  enTzCbcIntr=off  enTzDCAEVT1Intr=off  enTzDCAEVT2Intr=off  enTzDCBEVT1Intr=off  enTzDCBEVT2Intr=off  tzclrCBCLatch=Counter equals to zero (CTR=Zero)  ePWMxAforced=No action  ePWMxBforced=No action  DCAEVT1forced=No action  DCBEVT1forced=No action  DCAEVT2forced=No action  DCBEVT2forced=No action  dcah=Trip Zone 1 input (TZ1)  dcal=Trip Zone 2 input (TZ2)  dcbh=Trip Zone 1 input (TZ1)  dcbl=Trip Zone 2 input (TZ2)  dcah_type2=GPTRIP1SEL/(TZ1)  dcal_type2=GPTRIP2SEL/(TZ2)  dcbh_type2=GPTRIP1SEL/(TZ1)  dcbl_type2=GPTRIP2SEL/(TZ2)  gendcaevt1=Event disabled  gendcaevt2=Event disabled  gendcbevt1=Event disabled  gendcbevt2=Event disabled  dcaevt1src=DCAEVT1 with sync  dcaevt2src=DCAEVT2 with sync  dcbevt1src=DCBEVT1 with sync  dcbevt2src=DCBEVT2 with sync  pulsesel=Counter equals to zero (CTR=Zero)  blankinv=off  blankoffset=0  blankwidth=0  evsrcsel=Filtered version of DCAEVT1 (DCAEVT1FILT)  encape=off
  ePWM5 : c2802xlib/ePWM  PwmType=C2000_Type4  useModule=ePWM5  ePWMxLINKTBPRD=Not Linked  periodUnits=Clock cycles  timerSource=Specify via dialog  timerPeriod_clk=target.PWM_Counter_Period  timerPeriod_sec=0.0001  tbshadow=Counter equals to zero  countingMode=Up-Down  phaseActiveEnable=Set counter to phase value specified via dialog  phaseDirection=Count down after sync  phaseActive=target.PWM_Counter_Period  synchronizationEnable=off  dcaevt1Sync=off  dcbevt1Sync=off  synchronizationOption=Pass through (EPWMxSYNCI or SWFSYNC)  dcbevt1SyncOut=off  dcaevt1SyncOut=off  cmpdSyncOut=off  cmpcSyncOut=off  cmpbSyncOut=off  zeroSyncOut=off  swfSyncOut=on  perSynchronizationOption=Counter equals to period (CTR=PRD)  clockPrescale=1  HSclockPrescale=1  enswap=off  ePWMxAStatus=on  ePWMxAactionLogic1=Do nothing  ePWMxAactionLogic2=Do nothing  ePWMxAactionLogic3=Clear  ePWMxAactionLogic4=Set  ePWMxAactionLogic5=Do nothing  ePWMxAactionLogic6=Do nothing  ePWMxACSFenable=off  ePWMxACSFvalue=Forcing disable  ePWMxASFreload=Zero  ePWMxBStatus=off  ePWMxBactionLogic1=Set  ePWMxBactionLogic2=Clear  ePWMxBactionLogic3=Do nothing  ePWMxBactionLogic4=Do nothing  ePWMxBactionLogic5=Clear  ePWMxBactionLogic6=Set  ePWMxBCSFenable=off  ePWMxBCSFvalue=Forcing disable  ePWMxBSFreload=Zero  ePWNxBOutWay=off  ePWMxLINKCMPA=Not Linked  CMPAUnits=Clock cycles  CMPASource=Input port  CMPAValue_per=50  CMPAValue_clk=floor(target.PWM_Counter_Period/2)  enCMPAshadow=Counter equals to zero (CTR=Zero)  ePWMxLINKCMPB=Not Linked  CMPBUnits=Clock cycles  CMPBSource=Specify via dialog  CMPBValue_per=50  CMPBValue_clk=floor(target.PWM_Counter_Period/2)  enCMPBshadow=Counter equals to zero (CTR=Zero)  ePWMxLINKCMPC=Not Linked  CMPCUnits=Clock cycles  CMPCSource=Specify via dialog  CMPCValue_per=50  CMPCValue_clk=32000  enCMPCshadow=Counter equals to zero (CTR=Zero)  ePWMxLINKCMPD=Not Linked  CMPDUnits=Clock cycles  CMPDSource=Specify via dialog  CMPDValue_per=50  CMPDValue_clk=32000  enCMPDshadow=Counter equals to zero (CTR=Zero)  enableDBePWMxA=on  enableDBePWMxB=on  enhalfcycle=off  DBpolarity=Active high complementary (AHC)  DBedgeDelay=Positive  DBSource_ePWMxA=ePWMxA  DBSource_ePWMxB=ePWMxA  DBPeriodUnits=Clock cycles  DBperiodSource=Specify via dialog  REDperiod=10  FEDperiod=10  REDperiod_sec=0  FEDperiod_sec=0  LoadModeDBRED=Immediate without using shadow  LoadModeDBFED=Immediate without using shadow  adcstartModuleA=off  adcrequestEventA=First event  adcstartEventA=Digital Compare Module A Event 1 start of conversion (DCAEVT1.soc)  adcstartEventA_type2=Counter equals to period (CTR=PRD)  adcstartModuleB=off  adcrequestEventB=First event  adcstartEventB=Counter equals to zero (CTR=Zero)  adcstartEventB_type2=Counter equals to zero (CTR=Zero)  intEn=off  intPrd=First event  intSel=Counter equals to zero (CTR=Zero)  intSel_type2=Counter equals to zero (CTR=Zero)  hrpe=off  enHRPWM=off  HRPWM_LoadMode=Counter equals to period (CTR=PRD)  HRPWM_CTLMode=Duty or Period control mode  HRPWM_EDGMode=Both edge  hrpeb=off  enHRPWMB=off  HRPWM_LoadModeB=Counter equals to zero (CTR=ZERO)  HRPWM_CTLModeB=Duty or Period control mode  HRPWM_EDGModeB=Both edge  enHRDBRED=off  enHRDBFED=off  enSFO=on  enautoconv=on  chopperEnable=off  chopperFrequency=1  chopperFirstwidth=1  chopperDuty=12.5%  tripZonesource=Specify via dialog  tzselOSHT1=off  tzselOSHT2=off  tzselOSHT3=off  tzselOSHT4=off  tzselOSHT5=off  tzselOSHT6=off  tzselOSHDCAEV1=off  tzselOSHDCBEV1=off  tzselCBC1=off  tzselCBC2=off  tzselCBC3=off  tzselCBC4=off  tzselCBC5=off  tzselCBC6=off  tzselCBCDCAEV2=off  tzselCBCDCBEV2=off  enTzOstIntr=off  enTzCbcIntr=off  enTzDCAEVT1Intr=off  enTzDCAEVT2Intr=off  enTzDCBEVT1Intr=off  enTzDCBEVT2Intr=off  tzclrCBCLatch=Counter equals to zero (CTR=Zero)  ePWMxAforced=No action  ePWMxBforced=No action  DCAEVT1forced=No action  DCBEVT1forced=No action  DCAEVT2forced=No action  DCBEVT2forced=No action  dcah=Trip Zone 1 input (TZ1)  dcal=Trip Zone 2 input (TZ2)  dcbh=Trip Zone 1 input (TZ1)  dcbl=Trip Zone 2 input (TZ2)  dcah_type2=GPTRIP1SEL/(TZ1)  dcal_type2=GPTRIP2SEL/(TZ2)  dcbh_type2=GPTRIP1SEL/(TZ1)  dcbl_type2=GPTRIP2SEL/(TZ2)  gendcaevt1=Event disabled  gendcaevt2=Event disabled  gendcbevt1=Event disabled  gendcbevt2=Event disabled  dcaevt1src=DCAEVT1 with sync  dcaevt2src=DCAEVT2 with sync  dcbevt1src=DCBEVT1 with sync  dcbevt2src=DCBEVT2 with sync  pulsesel=Counter equals to zero (CTR=Zero)  blankinv=off  blankoffset=0  blankwidth=0  evsrcsel=Filtered version of DCAEVT1 (DCAEVT1FILT)  encape=off
  ePWM6 : c2802xlib/ePWM  PwmType=C2000_Type4  useModule=ePWM6  ePWMxLINKTBPRD=Not Linked  periodUnits=Clock cycles  timerSource=Specify via dialog  timerPeriod_clk=target.PWM_Counter_Period  timerPeriod_sec=0.0001  tbshadow=Counter equals to zero  countingMode=Up-Down  phaseActiveEnable=Set counter to phase value specified via dialog  phaseDirection=Count down after sync  phaseActive=target.PWM_Counter_Period  synchronizationEnable=off  dcaevt1Sync=off  dcbevt1Sync=off  synchronizationOption=Pass through (EPWMxSYNCI or SWFSYNC)  dcbevt1SyncOut=off  dcaevt1SyncOut=off  cmpdSyncOut=off  cmpcSyncOut=off  cmpbSyncOut=off  zeroSyncOut=off  swfSyncOut=on  perSynchronizationOption=Counter equals to period (CTR=PRD)  clockPrescale=1  HSclockPrescale=1  enswap=off  ePWMxAStatus=on  ePWMxAactionLogic1=Do nothing  ePWMxAactionLogic2=Do nothing  ePWMxAactionLogic3=Clear  ePWMxAactionLogic4=Set  ePWMxAactionLogic5=Do nothing  ePWMxAactionLogic6=Do nothing  ePWMxACSFenable=off  ePWMxACSFvalue=Forcing disable  ePWMxASFreload=Zero  ePWMxBStatus=off  ePWMxBactionLogic1=Set  ePWMxBactionLogic2=Clear  ePWMxBactionLogic3=Do nothing  ePWMxBactionLogic4=Do nothing  ePWMxBactionLogic5=Clear  ePWMxBactionLogic6=Set  ePWMxBCSFenable=off  ePWMxBCSFvalue=Forcing disable  ePWMxBSFreload=Zero  ePWNxBOutWay=off  ePWMxLINKCMPA=Not Linked  CMPAUnits=Clock cycles  CMPASource=Input port  CMPAValue_per=50  CMPAValue_clk=floor(target.PWM_Counter_Period/2)  enCMPAshadow=Counter equals to zero (CTR=Zero)  ePWMxLINKCMPB=Not Linked  CMPBUnits=Clock cycles  CMPBSource=Specify via dialog  CMPBValue_per=50  CMPBValue_clk=floor(target.PWM_Counter_Period/2)  enCMPBshadow=Counter equals to zero (CTR=Zero)  ePWMxLINKCMPC=Not Linked  CMPCUnits=Clock cycles  CMPCSource=Specify via dialog  CMPCValue_per=50  CMPCValue_clk=32000  enCMPCshadow=Counter equals to zero (CTR=Zero)  ePWMxLINKCMPD=Not Linked  CMPDUnits=Clock cycles  CMPDSource=Specify via dialog  CMPDValue_per=50  CMPDValue_clk=32000  enCMPDshadow=Counter equals to zero (CTR=Zero)  enableDBePWMxA=on  enableDBePWMxB=on  enhalfcycle=off  DBpolarity=Active high complementary (AHC)  DBedgeDelay=Positive  DBSource_ePWMxA=ePWMxA  DBSource_ePWMxB=ePWMxA  DBPeriodUnits=Clock cycles  DBperiodSource=Specify via dialog  REDperiod=10  FEDperiod=10  REDperiod_sec=0  FEDperiod_sec=0  LoadModeDBRED=Immediate without using shadow  LoadModeDBFED=Immediate without using shadow  adcstartModuleA=off  adcrequestEventA=First event  adcstartEventA=Digital Compare Module A Event 1 start of conversion (DCAEVT1.soc)  adcstartEventA_type2=Counter equals to period (CTR=PRD)  adcstartModuleB=off  adcrequestEventB=First event  adcstartEventB=Counter equals to zero (CTR=Zero)  adcstartEventB_type2=Counter equals to zero (CTR=Zero)  intEn=off  intPrd=First event  intSel=Counter equals to zero (CTR=Zero)  intSel_type2=Counter equals to zero (CTR=Zero)  hrpe=off  enHRPWM=off  HRPWM_LoadMode=Counter equals to period (CTR=PRD)  HRPWM_CTLMode=Duty or Period control mode  HRPWM_EDGMode=Both edge  hrpeb=off  enHRPWMB=off  HRPWM_LoadModeB=Counter equals to zero (CTR=ZERO)  HRPWM_CTLModeB=Duty or Period control mode  HRPWM_EDGModeB=Both edge  enHRDBRED=off  enHRDBFED=off  enSFO=on  enautoconv=on  chopperEnable=off  chopperFrequency=1  chopperFirstwidth=1  chopperDuty=12.5%  tripZonesource=Specify via dialog  tzselOSHT1=off  tzselOSHT2=off  tzselOSHT3=off  tzselOSHT4=off  tzselOSHT5=off  tzselOSHT6=off  tzselOSHDCAEV1=off  tzselOSHDCBEV1=off  tzselCBC1=off  tzselCBC2=off  tzselCBC3=off  tzselCBC4=off  tzselCBC5=off  tzselCBC6=off  tzselCBCDCAEV2=off  tzselCBCDCBEV2=off  enTzOstIntr=off  enTzCbcIntr=off  enTzDCAEVT1Intr=off  enTzDCAEVT2Intr=off  enTzDCBEVT1Intr=off  enTzDCBEVT2Intr=off  tzclrCBCLatch=Counter equals to zero (CTR=Zero)  ePWMxAforced=No action  ePWMxBforced=No action  DCAEVT1forced=No action  DCBEVT1forced=No action  DCAEVT2forced=No action  DCBEVT2forced=No action  dcah=Trip Zone 1 input (TZ1)  dcal=Trip Zone 2 input (TZ2)  dcbh=Trip Zone 1 input (TZ1)  dcbl=Trip Zone 2 input (TZ2)  dcah_type2=GPTRIP1SEL/(TZ1)  dcal_type2=GPTRIP2SEL/(TZ2)  dcbh_type2=GPTRIP1SEL/(TZ1)  dcbl_type2=GPTRIP2SEL/(TZ2)  gendcaevt1=Event disabled  gendcaevt2=Event disabled  gendcbevt1=Event disabled  gendcbevt2=Event disabled  dcaevt1src=DCAEVT1 with sync  dcaevt2src=DCAEVT2 with sync  dcbevt1src=DCBEVT1 with sync  dcbevt2src=DCBEVT2 with sync  pulsesel=Counter equals to zero (CTR=Zero)  blankinv=off  blankoffset=0  blankwidth=0  evsrcsel=Filtered version of DCAEVT1 (DCAEVT1FILT)  encape=off
  stop : Constant  Value=0  OutDataTypeStr=uint16
  DutyCycles : Outport  VectorParamsAs1DForOutWhenUnconnected=off
  wires:
  Demux1/3 -> ePWM6/1  "PWM_C"
  Scale_to_PWM_Counter_PRD/1 -> Switch1/1
  Mux2/1 -> Switch1/3
  stop/1 -> Mux2/3, Mux2/2, Mux2/1
  Demux/4 -> Switch1/2, NOT/1, Switch/1  "Active high logic for inverter enable"
  Inverter Signals/1 -> Demux/1
  Demux1/2 -> ePWM5/1  "PWM_B"
  Switch1/1 -> Demux1/1
  Demux1/1 -> ePWM4/1  "PWM_A"
  Mux/1 -> Scale_to_PWM_Counter_PRD/1  "PWM Duty Cycles"
  Ground/1 -> Mux1/1
  Ground1/1 -> Mux1/3
  Ground2/1 -> Mux1/2
  Mux1/1 -> DutyCycles/1
  Demux/1 -> Mux/1
  Demux/2 -> Mux/2
  Demux/3 -> Mux/3
  Constant/1 -> Switch/2
  NOT/1 -> Switch/3  "Active low logic for inverter enable"
  Switch/1 -> Inverter2 Enable/1

== system FOCwithLOAD/Motor2 Torque control/Inverter/Simulation ==
  Inverter Signals : Inport
  Data Type Duplicate : DataTypeDuplicate
  Demux : Demux
  Mux : Mux  Inputs=3
  Mux2 : Mux  Inputs=3
  Switch1 : Switch  Threshold=0.5  RndMeth=Simplest  SaturateOnIntegerOverflow=off  InputSameDT=off
  stop : Constant  Value=0  OutDataTypeStr=Inherit: Inherit via back propagation
  DutyCycles : Outport  VectorParamsAs1DForOutWhenUnconnected=off
  wires:
  stop/1 -> Data Type Duplicate/2, Mux2/1, Mux2/3, Mux2/2
  Mux2/1 -> Switch1/3
  Switch1/1 -> DutyCycles/1
  Inverter Signals/1 -> Demux/1
  Demux/4 -> Switch1/2  "PWM Enable"
  Mux/1 -> Data Type Duplicate/1, Switch1/1  "PWM Duty Cycles"
  Demux/1 -> Mux/1
  Demux/2 -> Mux/2
  Demux/3 -> Mux/3

== system FOCwithLOAD/Serial Receive/Parse SCI Rx/Data_Conditioning_Rx ==
  Rx : Inport
  Data_Type_Fixed_Point : Subsystem  VariantControl=~isequal(dataType, 'single')
  Data_Type_Float : Subsystem  VariantControl=isequal(dataType, 'single')
  Desired Speed : Outport
  Out2 : Outport  Port=2
  Desired torque : Outport  Port=3

== system FOCwithLOAD/Serial Receive/Parse SCI Rx/unParse ==
  Data : Inport
  Bitwise Operator : simulink/Logic and Bit Operations/Bitwise Operator  logicop=AND  UseBitMask=on  BitMask=hex2dec('0001')  BitMaskRealWorld=Stored Integer
  Bitwise Operator1 : simulink/Logic and Bit Operations/Bitwise Operator  logicop=AND  UseBitMask=on  BitMask=hex2dec('00F0')  BitMaskRealWorld=Stored Integer
  Bitwise Operator3 : simulink/Logic and Bit Operations/Bitwise Operator  logicop=AND  UseBitMask=on  BitMask=hex2dec('000C')  BitMaskRealWorld=Stored Integer
  Data Type Conversion3 : DataTypeConversion  OutDataTypeStr=boolean  RndMeth=Simplest  SaturateOnIntegerOverflow=off
  Data Type Conversion4 : DataTypeConversion  OutDataTypeStr=uint16  RndMeth=Simplest  SaturateOnIntegerOverflow=off
  Shift Arithmetic1 : ArithShift  BitShiftNumber=4
  Shift Arithmetic2 : ArithShift  BitShiftNumber=2
  Enable_PWM : Outport
  Debug_signals : Outport  Port=2
  CalMode : Outport  Port=3
  wires:
  Bitwise Operator1/1 -> Shift Arithmetic1/1
  Bitwise Operator/1 -> Data Type Conversion3/1
  Data Type Conversion4/1 -> Debug_signals/1
  Shift Arithmetic1/1 -> Data Type Conversion4/1
  Data Type Conversion3/1 -> Enable_PWM/1
  ? -> ?
  ? -> ?
  ? -> ?
  ? -> ?
  Bitwise Operator3/1 -> Shift Arithmetic2/1
  Shift Arithmetic2/1 -> CalMode/1
  Data/1 -> Bitwise Operator3/1, Bitwise Operator/1, Bitwise Operator1/1

== system FOCwithLOAD/Serial Receive/Serial Receive/Serial Rx ==
  Data_Type_Fixed_Point : Subsystem  VariantControl=~isequal(dataType, 'single')
  Data_Type_Float : Subsystem  VariantControl=isequal(dataType, 'single')
  Rx : Outport

== system FOCwithLOAD/Serial Receive/Signal Packing/Data_Conditioning_Tx ==
  Speedref : Inport
  In2 : Inport  Port=2
  IqRef : Inport  Port=3
  Data_Type_Fixed_Point : Subsystem  VariantControl=~isequal(dataType, 'single')
  Data_Type_Float : Subsystem  VariantControl=isequal(dataType, 'single')
  Data : Outport

== system FOCwithLOAD/Serial Receive/Signal Packing/Parse ==
  Enable_PWM : Inport
  Debug_signals : Inport  Port=2
  Bitwise Operator : simulink/Logic and Bit Operations/Bitwise Operator  logicop=AND  UseBitMask=on  BitMask=hex2dec('0003')  BitMaskRealWorld=Stored Integer
  Bitwise Operator1 : simulink/Logic and Bit Operations/Bitwise Operator  logicop=AND  UseBitMask=on  BitMask=hex2dec('00F0')  BitMaskRealWorld=Stored Integer
  RunEnableSim : Constant  OutDataTypeStr=uint16
  Shift Arithmetic1 : ArithShift  BitShiftNumber=-4
  ShiftCal : ArithShift  BitShiftNumber=-2
  Sum : Sum  Inputs=+++
  Data : Outport
  wires:
  Debug_signals/1 -> Shift Arithmetic1/1
  Sum/1 -> Data/1
  Shift Arithmetic1/1 -> Bitwise Operator1/1
  Enable_PWM/1 -> Bitwise Operator/1
  Bitwise Operator1/1 -> Sum/2
  ShiftCal/1 -> Sum/3
  Bitwise Operator/1 -> ShiftCal/1
  RunEnableSim/1 -> Sum/1

== system FOCwithLOAD/Hardware Init/Variant Subsystem/Code Generation/DRV Enable ==
  note: Enable inverter1 8323
  note: Enable PMSM2 inverter2 8323
  Constant : Constant  Value=inverter.EnableLogic
  Constant1 : Constant  Value=inverter2.EnableLogic
  Digital Output : c2837xDlib/Digital Output  Priority=10  GPIO_Number=GPIO24~GPIO31  GPIO_Bit0=on  GPIO_BIT0_Toggle=off  GPIO_Bit1=off  GPIO_BIT1_Toggle=off  GPIO_Bit2=off  GPIO_BIT2_Toggle=off  GPIO_Bit3=off  GPIO_BIT3_Toggle=off  GPIO_Bit4=off  GPIO_BIT4_Toggle=off  GPIO_Bit5=off  GPIO_BIT5_Toggle=off  GPIO_Bit6=off  GPIO_BIT6_Toggle=off  GPIO_Bit7=off  GPIO_BIT7_Toggle=off
  Digital Output1 : c2837xDlib/Digital Output  Priority=10  GPIO_Number=GPIO8~GPIO15  GPIO_Bit0=off  GPIO_BIT0_Toggle=off  GPIO_Bit1=off  GPIO_BIT1_Toggle=off  GPIO_Bit2=off  GPIO_BIT2_Toggle=off  GPIO_Bit3=off  GPIO_BIT3_Toggle=off  GPIO_Bit4=off  GPIO_BIT4_Toggle=off  GPIO_Bit5=off  GPIO_BIT5_Toggle=off  GPIO_Bit6=on  GPIO_BIT6_Toggle=off  GPIO_Bit7=off  GPIO_BIT7_Toggle=off
  Inverter Enable : Constant  OutDataTypeStr=uint16  SampleTime=-1
  Inverter Enable1 : Constant  OutDataTypeStr=uint16  SampleTime=-1
  NOT : Logic  Operator=NOT  IconShape=distinctive  AllPortsSameDT=off  OutDataTypeStr=boolean
  NOT1 : Logic  Operator=NOT  IconShape=distinctive  AllPortsSameDT=off  OutDataTypeStr=boolean
  Switch : Switch  Criteria=u2 > Threshold  SaturateOnIntegerOverflow=off  InputSameDT=off
  Switch1 : Switch  Criteria=u2 > Threshold  SaturateOnIntegerOverflow=off  InputSameDT=off
  wires:
  Inverter Enable/1 -> Switch/1, NOT/1  "Active high logic for inverter enable"
  Constant/1 -> Switch/2
  Switch/1 -> Digital Output/1
  NOT/1 -> Switch/3  "Active low logic for inverter enable"
  Inverter Enable1/1 -> Switch1/1, NOT1/1  "Active high logic for inverter enable"
  Switch1/1 -> Digital Output1/1
  Constant1/1 -> Switch1/2
  NOT1/1 -> Switch1/3  "Active low logic for inverter enable"

== system FOCwithLOAD/Motor1 Speed control/Control_System/Closed Loop Control1/Angle Compensate ==
  note: 已经被归一化0-1
  note: [(SpeedSample / 60)* 3] * Ts
  note: 高速运行时角度传感器读取存在延迟，
      | 在Ts的采样周期内，电机又转了
  ThetaeSample : Inport
  SpeedSample : Inport  Port=2
  Add : Sum
  Gain : Gain  Gain=pmsm.p/(60*speedRPM2mmps)*Ts
  Thetae : Outport
  wires:
  Gain/1 -> Add/2
  Add/1 -> Thetae/1
  SpeedSample/1 -> Gain/1
  ThetaeSample/1 -> Add/1
